simulink model "COMPONENT_POS_CMD"  (R2026b)
settings: Solver=VariableStepAuto
libraries: simulink_extras x3
settings Model: Creator=bhorton  LastModifiedBy=bhorton

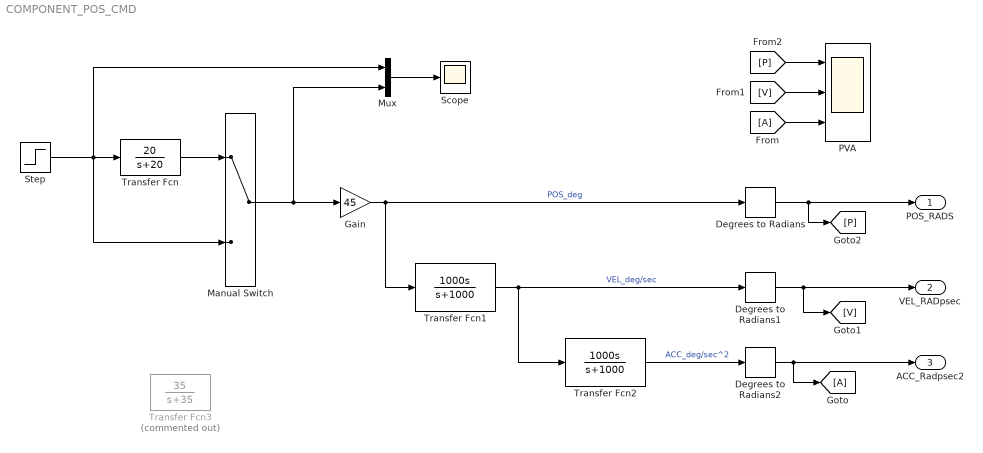
== system COMPONENT_POS_CMD ==
  Degrees to Radians : simulink_extras/Transformations/Degrees to Radians
  Degrees to Radians1 : simulink_extras/Transformations/Degrees to Radians
  Degrees to Radians2 : simulink_extras/Transformations/Degrees to Radians
  From : From
  Gain : Gain  Gain=45
  Goto : Goto
  Manual Switch : ManualSwitch
  Mux : Mux  Inputs=2
  PVA : Scope  NumInputPorts=3
      settings: ActiveDisplayYMinimum=-0.098174770424681007  ActiveDisplayYMaximum=0.88357293382212931  DataLoggingVariableName=ScopeData4
  Scope : Scope
      settings: ActiveDisplayYMinimum=-0.0343389396209719  ActiveDisplayYMaximum=1.0137019750266969
  Step : Step  SampleTime=0
  Transfer Fcn : TransferFcn  Numerator=[20]  Denominator=[1 20]
  Transfer Fcn1 : TransferFcn  Numerator=[1000 0]  Denominator=[1 1000]
  Transfer Fcn2 : TransferFcn  Numerator=[1000 0]  Denominator=[1 1000]
  Transfer Fcn3 : TransferFcn  Commented=on  Numerator=[35]  Denominator=[1 35]
  POS_RADS : Outport
  VEL_RADpsec : Outport  Port=2
  ACC_Radpsec2 : Outport  Port=3
  wires:
  Gain/1 -> Degrees to Radians/1, Transfer Fcn1/1  "POS_deg"
  Step/1 -> Manual Switch/2, Mux/1, Transfer Fcn/1
  Mux/1 -> Scope/1
  Degrees to Radians/1 -> POS_RADS/1, [P]
  Manual Switch/1 -> Mux/2, Gain/1
  Degrees to Radians1/1 -> VEL_RADpsec/1, [V]
  Transfer Fcn1/1 -> Degrees to Radians1/1, Transfer Fcn2/1  "VEL_deg/sec"
  Degrees to Radians2/1 -> ACC_Radpsec2/1, Goto/1
  Transfer Fcn2/1 -> Degrees to Radians2/1  "ACC_deg/sec^2"
  [P] -> PVA/1
  [V] -> PVA/2
  From/1 -> PVA/3
  Transfer Fcn/1 -> Manual Switch/1
